simulink model "sfbg_lqr_occ_"  (R2024b)
settings: Solver=FixedStepAuto  StartTime=0.0  StopTime=Ts  FixedStep=Ts  RelTol=1e-3
InitFcn:
  | load('.\data_smk_\fbg_controller_parameters.mat')
settings Model: Creator=rmrane  LastModifiedBy=vreyesdreke
settings OptimizationCC: DefaultParameterBehavior=Inlined  EnhancedBackFolding=on  PassReuseOutputArgsAs=Individual arguments  ZeroExternalMemoryAtStartup=off  ZeroInternalMemoryAtStartup=off  OptimizeBlockOrder=speed  DifferentSizesBufferReuse=on  OptimizationCustomize=off  EfficientTunableParamExpr=on
settings DebuggingCC: ParameterTunabilityLossMsg=error
settings SFSimCC: MATLABDynamicMemAlloc=off
settings RTWCC: Description=Embedded Coder  SystemTargetFile=ert.tlc  TemplateMakefile=ert_default_tmf
settings CodeAppCC: GenerateComments=off  IgnoreCustomStorageClasses=off  OperatorAnnotations=on  SimulinkDataObjDesc=on  SFDataObjDesc=on  CustomSymbolStrType=$N$R$M  SimulinkBlockComments=off  InternalIdentifier=Classic
settings ERTTargetCC: GenerateSampleERTMain=on  SupportAbsoluteTime=off  SupportNonFinite=off  SupportComplex=off  ERTCustomFileTemplate=example_file_process.tlc  ConvertIfToSwitch=off  SuppressUnreachableDefaultCases=off  EnableSignedLeftShifts=off  EnableSignedRightShifts=off  DynamicArrayContainerType=coder::array

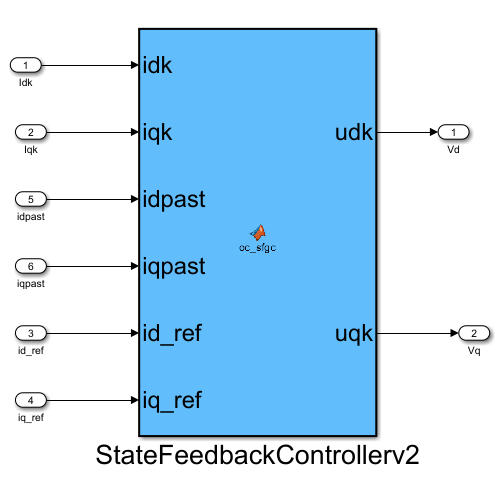
[thumbnail: Simulink's stored preview of the top-level diagram]
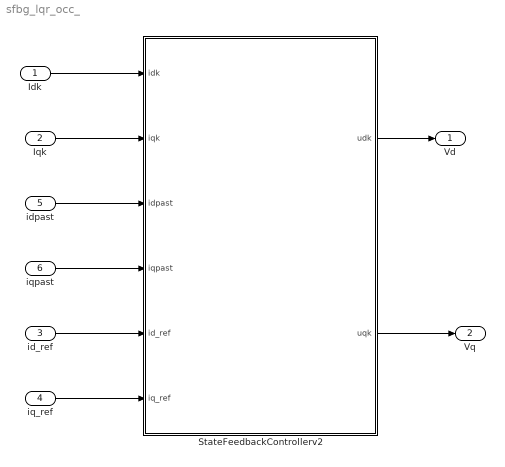
== system sfbg_lqr_occ_ ==
  Idk : Inport
  Iqk : Inport  Port=2
  id_ref : Inport  Port=3
  iq_ref : Inport  Port=4
  idpast : Inport  Port=5
  iqpast : Inport  Port=6
  StateFeedbackControllerv2 : MATLAB Function  TreatAsAtomicUnit=on
  Vd : Outport
  Vq : Outport  Port=2
  wires:
  Idk/1 -> StateFeedbackControllerv2/1(idk)
  Iqk/1 -> StateFeedbackControllerv2/2(iqk)
  idpast/1 -> StateFeedbackControllerv2/3(idpast)
  iqpast/1 -> StateFeedbackControllerv2/4(iqpast)
  StateFeedbackControllerv2/1(udk) -> Vd/1
  StateFeedbackControllerv2/2(uqk) -> Vq/1
  id_ref/1 -> StateFeedbackControllerv2/5(id_ref)
  iq_ref/1 -> StateFeedbackControllerv2/6(iq_ref)

== matlab function sfbg_lqr_occ_/StateFeedbackControllerv2 ==
  settings: updateMethod=DISCRETE  sampleTime=Ts
  data: idk input size=1; udk output size=1; uqk output size=1; iqk input size=1; idpast input size=1; iqpast input size=1; id_ref input size=1; iq_ref input size=1
function [udk,uqk] = oc_sfgc(idk, iqk,idpast, iqpast,id_ref,iq_ref)
    % oc_sfc(idk, iqk,id_ref,iq_ref) feedforward controller gain.
    m_ss = coder.load('.\data_smk_\fbg_controller_parameters.mat','-mat','-regexp','Kfbg_LQR');
    ekvec = [(idk-idpast), (iqk-iqpast),idk,iqk]'-[0,0,id_ref,iq_ref]';
    uk = m_ss.Kfbg_LQR*ekvec;
    udk = uk(1);
    uqk = uk(2);
end
